simulink model "WaveStar"  (R2020b)
settings: Solver=ode4  StartTime=0  StopTime=141.2  FixedStep=0.001  MaxStep=0.001  RelTol=1e-3  EnableMultiTasking=on
values from neighbouring files (symbols this model uses):
  cc = 10.0    (= 10)    [controller_init.m]
  kc = 0    [controller_init.m]
  L_AB = 0.412    [controller_init.m]
  L_AC = 0.2    [controller_init.m]
  mc = 0    [controller_init.m]
  McSat = inf    [controller_init.m]
  simu = simulationClass()    [wecSimInputFile.m]
  xPcTs = 0.001    [controller_init.m]
undefined symbols (not defined in the file or in its folder): body, constraint, geometry, HPfreq, hydroData, LPfreq, pto, X, Y, Z
libraries: nesl_utility x36, sm_lib x26, WECSim_Lib_Body_Elements x5, simulink x2, WECSim_Lib_Constraints x2, WECSim_Lib_Frames x1
(part 2 of 2)

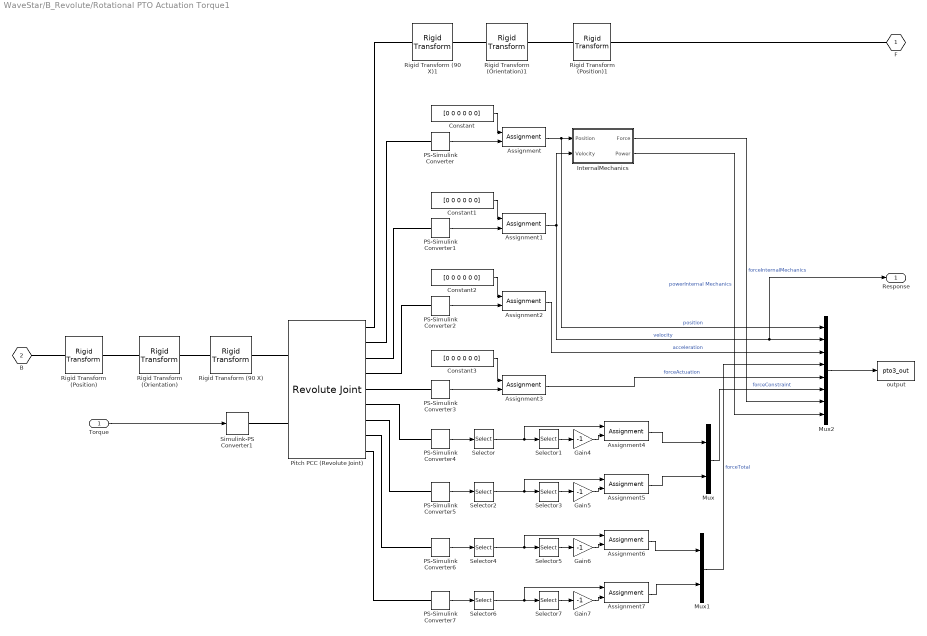
== system WaveStar/B_Revolute/Rotational PTO Actuation Torque1 ==
  Torque : Inport
  "Assignment " : Assignment  IndexOptions=Index vector (dialog)  Indices=5  OutputSizes=1
  Assignment1 : Assignment  IndexOptions=Index vector (dialog)  Indices=5  OutputSizes=1
  Assignment2 : Assignment  IndexOptions=Index vector (dialog)  Indices=5  OutputSizes=1
  Assignment3 : Assignment  IndexOptions=Index vector (dialog)  Indices=5  OutputSizes=1
  Assignment{4..7} (4 alike) : Assignment  DiagnosticForDimensions=Warning  IndexOptions=Index vector (dialog)  Indices=3  OutputSizes=1
  Constant{,1..3} (4 alike) : Constant  Value=[0 0 0 0 0 0]
  Gain{4..7} (4 alike) : Gain  Gain=-1
  InternalMechanics : Subsystem
  Mux : Mux  Inputs=2
  Mux1 : Mux  Inputs=2
  Mux2 : Mux  Inputs=8
  PS-Simulink Converter{,1..7} (8 alike) : nesl_utility/PS-Simulink Converter  PhysicalDomain=network_engine_domain  SubClassName=ps_output  LeftPortType=input  RightPortType=output  PseudoPeriodic=off  Frequencies=[]  VectorFormat=1-D array  Unit=1  AffineConversion=off
  Pitch PCC (Revolute Joint) : sm_lib/Joints/Revolute Joint  JointMode=Normal  SenseConstraintForce=on  SenseConstraintForceX=off  SenseConstraintForceY=off  SenseConstraintForceZ=off  SenseConstraintTorque=on  SenseConstraintTorqueX=off  SenseConstraintTorqueY=off  SenseConstraintTorqueZ=off  SenseTotalForce=on  SenseTotalForceX=off  SenseTotalForceY=off  SenseTotalForceZ=off  SenseTotalTorque=on  SenseTotalTorqueX=off  SenseTotalTorqueY=off  SenseTotalTorqueZ=off  CompositeWrenchDir=BaseOnFollower  CompositeWrenchFrame=BaseFrame  EquilibriumPosition=0  EquilibriumPositionUnits=deg  SpringStiffness=pto.stiffness  SpringStiffnessUnits=N*m/rad  DampingCoefficient=pto.damping  DampingCoefficientUnits=N*m/(rad/s)  TorqueActuationMode=InputTorque  MotionActuationMode=ComputedMotion  SensePosition=on  SenseVelocity=on  SenseAcceleration=on  SenseTorqueForce=on  SenseLowerLimitTorqueForce=off  SenseUpperLimitTorqueForce=off  LowerLimitSpecify=off  LowerLimitBound=-90  LowerLimitBoundUnits=deg  LowerLimitStiffness=1e4  LowerLimitStiffnessUnits=N*m/deg  LowerLimitDamping=10  LowerLimitDampingUnits=N*m/(deg/s)  LowerLimitTransitionRegionWidth=0.1  LowerLimitTransitionRegionWidthUnits=deg  UpperLimitSpecify=off  UpperLimitBound=90  UpperLimitBoundUnits=deg  UpperLimitStiffness=1e4  UpperLimitStiffnessUnits=N*m/deg  UpperLimitDamping=10  UpperLimitDampingUnits=N*m/(deg/s)  UpperLimitTransitionRegionWidth=0.1  UpperLimitTransitionRegionWidthUnits=deg  PositionTargetSpecify=off  PositionTargetPriority=High  PositionTargetValue=0  PositionTargetValueUnits=deg  VelocityTargetSpecify=off  VelocityTargetPriority=High  VelocityTargetValue=0  VelocityTargetValueUnits=deg/s
  Rigid Transform (Position) : sm_lib/Frames and Transforms/Rigid Transform  TranslationMethod=Cartesian  TranslationStandardOffset=0  TranslationStandardOffsetUnits=m  TranslationStandardAxis=+Z  TranslationCartesianOffset=pto.initial.displacement + pto.location  TranslationCartesianOffsetUnits=m  TranslationROffset=0  TranslationROffsetUnits=m  TranslationZOffset=0  TranslationZOffsetUnits=m  TranslationThetaOffset=0  TranslationThetaOffsetUnits=deg  RotationMethod=None  RotationAngleUnits=rad  RotationStandardAxis=+Y  RotationAngle=0  RotationArbitraryAxis=[0 1 0]  FollAlignAxisA=+X  BaseAlignAxisA=+Y  FollAlignAxisB=+Y  BaseAlignAxisB=+Z  RotationSequenceAxes=FollowerAxes  RotationSequence=XYX  RotationSequenceAngles=[0 0 0]  RotationSequenceAnglesUnits=deg  RotationMatrix=[1 0 0; 0 1 0; 0 0 1]  Quaternion=[1 0 0 0]
  Rigid Transform (Position)1 : sm_lib/Frames and Transforms/Rigid Transform  TranslationMethod=Cartesian  TranslationStandardOffset=0  TranslationStandardOffsetUnits=m  TranslationStandardAxis=+Z  TranslationCartesianOffset=pto.initial.displacement + pto.location  TranslationCartesianOffsetUnits=m  TranslationROffset=0  TranslationROffsetUnits=m  TranslationZOffset=0  TranslationZOffsetUnits=m  TranslationThetaOffset=0  TranslationThetaOffsetUnits=deg  RotationMethod=None  RotationAngleUnits=rad  RotationStandardAxis=+Y  RotationAngle=0  RotationArbitraryAxis=[0 1 0]  FollAlignAxisA=+X  BaseAlignAxisA=+Y  FollAlignAxisB=+Y  BaseAlignAxisB=+Z  RotationSequenceAxes=FollowerAxes  RotationSequence=XYX  RotationSequenceAngles=[0 0 0]  RotationSequenceAnglesUnits=deg  RotationMatrix=[1 0 0; 0 1 0; 0 0 1]  Quaternion=[1 0 0 0]
  Rigid Transform (90 X) : sm_lib/Frames and Transforms/Rigid Transform  TranslationMethod=None  TranslationStandardOffset=0  TranslationStandardOffsetUnits=m  TranslationStandardAxis=+Z  TranslationCartesianOffset=0  TranslationCartesianOffsetUnits=m  TranslationROffset=0  TranslationROffsetUnits=m  TranslationZOffset=0  TranslationZOffsetUnits=m  TranslationThetaOffset=0  TranslationThetaOffsetUnits=deg  RotationMethod=StandardAxis  RotationAngleUnits=deg  RotationStandardAxis=+X  RotationAngle=-90  RotationArbitraryAxis=[0 1 0]  FollAlignAxisA=+X  BaseAlignAxisA=+Y  FollAlignAxisB=+Y  BaseAlignAxisB=+Z  RotationSequenceAxes=FollowerAxes  RotationSequence=XYX  RotationSequenceAngles=[0 0 0]  RotationSequenceAnglesUnits=deg  RotationMatrix=[1 0 0; 0 1 0; 0 0 1]  Quaternion=[1 0 0 0]
  Rigid Transform (90 X)1 : sm_lib/Frames and Transforms/Rigid Transform  TranslationMethod=None  TranslationStandardOffset=0  TranslationStandardOffsetUnits=m  TranslationStandardAxis=+Z  TranslationCartesianOffset=0  TranslationCartesianOffsetUnits=m  TranslationROffset=0  TranslationROffsetUnits=m  TranslationZOffset=0  TranslationZOffsetUnits=m  TranslationThetaOffset=0  TranslationThetaOffsetUnits=deg  RotationMethod=StandardAxis  RotationAngleUnits=deg  RotationStandardAxis=+X  RotationAngle=-90  RotationArbitraryAxis=[0 1 0]  FollAlignAxisA=+X  BaseAlignAxisA=+Y  FollAlignAxisB=+Y  BaseAlignAxisB=+Z  RotationSequenceAxes=FollowerAxes  RotationSequence=XYX  RotationSequenceAngles=[0 0 0]  RotationSequenceAnglesUnits=deg  RotationMatrix=[1 0 0; 0 1 0; 0 0 1]  Quaternion=[1 0 0 0]
  Rigid Transform (Orientation) : sm_lib/Frames and Transforms/Rigid Transform  TranslationMethod=None  TranslationStandardOffset=0  TranslationStandardOffsetUnits=m  TranslationStandardAxis=+Z  TranslationCartesianOffset=0  TranslationCartesianOffsetUnits=m  TranslationROffset=0  TranslationROffsetUnits=m  TranslationZOffset=0  TranslationZOffsetUnits=m  TranslationThetaOffset=0  TranslationThetaOffsetUnits=deg  RotationMethod=RotationMatrix  RotationAngleUnits=rad  RotationStandardAxis=+Y  RotationAngle=0  RotationArbitraryAxis=[0 1 0]  FollAlignAxisA=+X  BaseAlignAxisA=+Y  FollAlignAxisB=+Y  BaseAlignAxisB=+Z  RotationSequenceAxes=FollowerAxes  RotationSequence=XYX  RotationSequenceAngles=[0 0 0]  RotationSequenceAnglesUnits=deg  RotationMatrix=pto.orientation.rotationMatrix  Quaternion=[1 0 0 0]
  Rigid Transform (Orientation)1 : sm_lib/Frames and Transforms/Rigid Transform  TranslationMethod=None  TranslationStandardOffset=0  TranslationStandardOffsetUnits=m  TranslationStandardAxis=+Z  TranslationCartesianOffset=0  TranslationCartesianOffsetUnits=m  TranslationROffset=0  TranslationROffsetUnits=m  TranslationZOffset=0  TranslationZOffsetUnits=m  TranslationThetaOffset=0  TranslationThetaOffsetUnits=deg  RotationMethod=RotationMatrix  RotationAngleUnits=rad  RotationStandardAxis=+Y  RotationAngle=0  RotationArbitraryAxis=[0 1 0]  FollAlignAxisA=+X  BaseAlignAxisA=+Y  FollAlignAxisB=+Y  BaseAlignAxisB=+Z  RotationSequenceAxes=FollowerAxes  RotationSequence=XYX  RotationSequenceAngles=[0 0 0]  RotationSequenceAnglesUnits=deg  RotationMatrix=pto.orientation.rotationMatrix  Quaternion=[1 0 0 0]
  Selector{,2,4,6} (4 alike) : Selector  InputPortWidth=3  IndexOptions=Index vector (dialog)  Indices=[1 3 2]  OutputSizes=1
  Selector{1,3,5,7} (4 alike) : Selector  InputPortWidth=3  IndexOptions=Index vector (dialog)  Indices=[3]  OutputSizes=1
  Simulink-PS Converter1 : nesl_utility/Simulink-PS Converter  PhysicalDomain=network_engine_domain  SubClassName=ps_input  LeftPortType=input  RightPortType=output  PseudoPeriodic=off  Frequencies=[]  NoiseDistribution=none  NoiseParameters=[]  Unit=1  AffineConversion=off  FilteringAndDerivatives=zero  SimscapeFilterOrder=1  InputFilterTimeConstant=0.001  UdotUserProvided=1
  output : ToWorkspace  VariableName=pto3_out  SaveFormat=Structure With Time  SampleTime=-1
      settings: Decimation=round(simu.dtOut/simu.dt,0)
  F : PMIOPort  Side=Right
  B : PMIOPort  Port=2  Side=Left
  Response : Outport  VectorParamsAs1DForOutWhenUnconnected=off
  wires:
  Torque/1 -> Simulink-PS Converter1/1
  "Assignment "/1 -> Mux2/1, InternalMechanics/1(Position)  "position"
  Assignment1/1 -> Response/1, Mux2/2, InternalMechanics/2(Velocity)  "velocity"
  Assignment2/1 -> Mux2/3  "acceleration"
  Selector2/1 -> Assignment5/1, Selector3/1
  Selector3/1 -> Gain5/1
  Gain5/1 -> Assignment5/2
  Selector/1 -> Assignment4/1, Selector1/1
  Selector1/1 -> Gain4/1
  Gain4/1 -> Assignment4/2
  Assignment5/1 -> Mux/2
  Assignment4/1 -> Mux/1
  Mux/1 -> Mux2/6  "forceConstraint"
  PS-Simulink Converter5/1 -> Selector2/1
  PS-Simulink Converter4/1 -> Selector/1
  Mux2/1 -> output/1
  Mux1/1 -> Mux2/4  "forceTotal"
  Selector6/1 -> Selector7/1, Assignment7/1
  Selector7/1 -> Gain7/1
  Gain7/1 -> Assignment7/2
  Selector4/1 -> Selector5/1, Assignment6/1
  Selector5/1 -> Gain6/1
  Gain6/1 -> Assignment6/2
  PS-Simulink Converter6/1 -> Selector4/1
  PS-Simulink Converter7/1 -> Selector6/1
  Assignment7/1 -> Mux1/2
  Assignment6/1 -> Mux1/1
  Constant/1 -> "Assignment "/1
  PS-Simulink Converter/1 -> "Assignment "/2
  Constant1/1 -> Assignment1/1
  PS-Simulink Converter1/1 -> Assignment1/2
  Constant2/1 -> Assignment2/1
  PS-Simulink Converter2/1 -> Assignment2/2
  Constant3/1 -> Assignment3/1
  PS-Simulink Converter3/1 -> Assignment3/2
  Assignment3/1 -> Mux2/5  "forceActuation"
  InternalMechanics/1(Force) -> Mux2/7  "forceInternalMechanics"
  InternalMechanics/2(Power) -> Mux2/8  "powerInternal Mechanics"
  connections:
  Rigid Transform (Position)1/LConn1 -- F/RConn1
  Rigid Transform (Position)/RConn1 -- Rigid Transform (Orientation)/LConn1
  Rigid Transform (Orientation)/RConn1 -- Rigid Transform (90 X)/LConn1
  Rigid Transform (Orientation)1/RConn1 -- Rigid Transform (90 X)1/LConn1
  Rigid Transform (Position)1/RConn1 -- Rigid Transform (Orientation)1/LConn1
  Rigid Transform (90 X)/RConn1 -- Pitch PCC (Revolute Joint)/LConn1
  Pitch PCC (Revolute Joint)/LConn2 -- Simulink-PS Converter1/RConn1
  Rigid Transform (Position)/LConn1 -- B/RConn1
  PS-Simulink Converter7/LConn1 -- Pitch PCC (Revolute Joint)/RConn9
  PS-Simulink Converter6/LConn1 -- Pitch PCC (Revolute Joint)/RConn8
  PS-Simulink Converter5/LConn1 -- Pitch PCC (Revolute Joint)/RConn7
  PS-Simulink Converter4/LConn1 -- Pitch PCC (Revolute Joint)/RConn6
  Pitch PCC (Revolute Joint)/RConn2 -- PS-Simulink Converter/LConn1
  Pitch PCC (Revolute Joint)/RConn3 -- PS-Simulink Converter1/LConn1
  PS-Simulink Converter2/LConn1 -- Pitch PCC (Revolute Joint)/RConn4
  PS-Simulink Converter3/LConn1 -- Pitch PCC (Revolute Joint)/RConn5
  Rigid Transform (90 X)1/RConn1 -- Pitch PCC (Revolute Joint)/RConn1

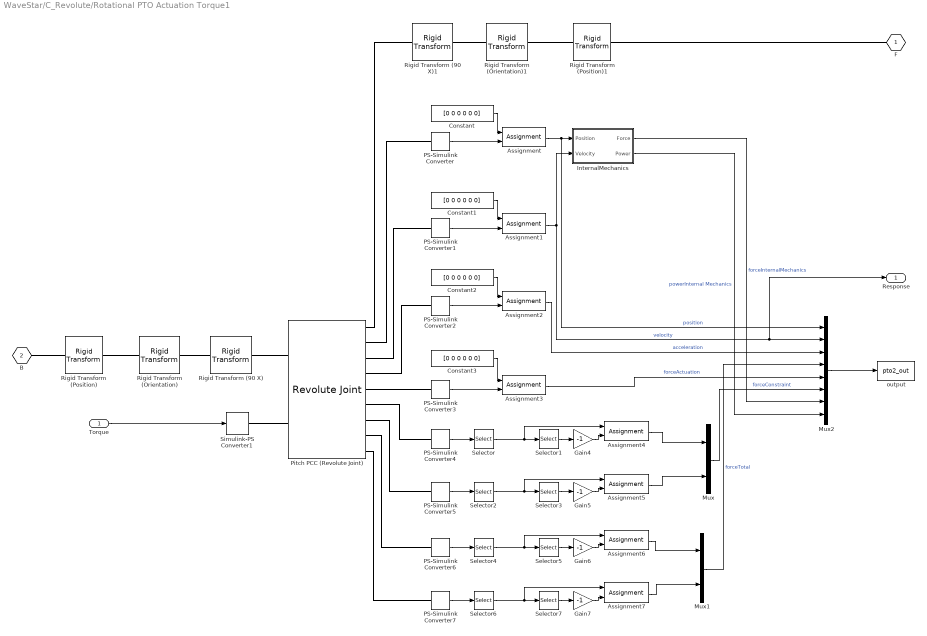
== system WaveStar/C_Revolute/Rotational PTO Actuation Torque1 ==
  Torque : Inport
  "Assignment " : Assignment  IndexOptions=Index vector (dialog)  Indices=5  OutputSizes=1
  Assignment1 : Assignment  IndexOptions=Index vector (dialog)  Indices=5  OutputSizes=1
  Assignment2 : Assignment  IndexOptions=Index vector (dialog)  Indices=5  OutputSizes=1
  Assignment3 : Assignment  IndexOptions=Index vector (dialog)  Indices=5  OutputSizes=1
  Assignment{4..7} (4 alike) : Assignment  DiagnosticForDimensions=Warning  IndexOptions=Index vector (dialog)  Indices=3  OutputSizes=1
  Constant{,1..3} (4 alike) : Constant  Value=[0 0 0 0 0 0]
  Gain{4..7} (4 alike) : Gain  Gain=-1
  InternalMechanics : Subsystem
  Mux : Mux  Inputs=2
  Mux1 : Mux  Inputs=2
  Mux2 : Mux  Inputs=8
  PS-Simulink Converter{,1..7} (8 alike) : nesl_utility/PS-Simulink Converter  PhysicalDomain=network_engine_domain  SubClassName=ps_output  LeftPortType=input  RightPortType=output  PseudoPeriodic=off  Frequencies=[]  VectorFormat=1-D array  Unit=1  AffineConversion=off
  Pitch PCC (Revolute Joint) : sm_lib/Joints/Revolute Joint  JointMode=Normal  SenseConstraintForce=on  SenseConstraintForceX=off  SenseConstraintForceY=off  SenseConstraintForceZ=off  SenseConstraintTorque=on  SenseConstraintTorqueX=off  SenseConstraintTorqueY=off  SenseConstraintTorqueZ=off  SenseTotalForce=on  SenseTotalForceX=off  SenseTotalForceY=off  SenseTotalForceZ=off  SenseTotalTorque=on  SenseTotalTorqueX=off  SenseTotalTorqueY=off  SenseTotalTorqueZ=off  CompositeWrenchDir=BaseOnFollower  CompositeWrenchFrame=BaseFrame  EquilibriumPosition=0  EquilibriumPositionUnits=deg  SpringStiffness=pto.stiffness  SpringStiffnessUnits=N*m/rad  DampingCoefficient=pto.damping  DampingCoefficientUnits=N*m/(rad/s)  TorqueActuationMode=InputTorque  MotionActuationMode=ComputedMotion  SensePosition=on  SenseVelocity=on  SenseAcceleration=on  SenseTorqueForce=on  SenseLowerLimitTorqueForce=off  SenseUpperLimitTorqueForce=off  LowerLimitSpecify=off  LowerLimitBound=-90  LowerLimitBoundUnits=deg  LowerLimitStiffness=1e4  LowerLimitStiffnessUnits=N*m/deg  LowerLimitDamping=10  LowerLimitDampingUnits=N*m/(deg/s)  LowerLimitTransitionRegionWidth=0.1  LowerLimitTransitionRegionWidthUnits=deg  UpperLimitSpecify=off  UpperLimitBound=90  UpperLimitBoundUnits=deg  UpperLimitStiffness=1e4  UpperLimitStiffnessUnits=N*m/deg  UpperLimitDamping=10  UpperLimitDampingUnits=N*m/(deg/s)  UpperLimitTransitionRegionWidth=0.1  UpperLimitTransitionRegionWidthUnits=deg  PositionTargetSpecify=off  PositionTargetPriority=High  PositionTargetValue=0  PositionTargetValueUnits=deg  VelocityTargetSpecify=off  VelocityTargetPriority=High  VelocityTargetValue=0  VelocityTargetValueUnits=deg/s
  Rigid Transform (Position) : sm_lib/Frames and Transforms/Rigid Transform  TranslationMethod=Cartesian  TranslationStandardOffset=0  TranslationStandardOffsetUnits=m  TranslationStandardAxis=+Z  TranslationCartesianOffset=pto.initial.displacement + pto.location  TranslationCartesianOffsetUnits=m  TranslationROffset=0  TranslationROffsetUnits=m  TranslationZOffset=0  TranslationZOffsetUnits=m  TranslationThetaOffset=0  TranslationThetaOffsetUnits=deg  RotationMethod=None  RotationAngleUnits=rad  RotationStandardAxis=+Y  RotationAngle=0  RotationArbitraryAxis=[0 1 0]  FollAlignAxisA=+X  BaseAlignAxisA=+Y  FollAlignAxisB=+Y  BaseAlignAxisB=+Z  RotationSequenceAxes=FollowerAxes  RotationSequence=XYX  RotationSequenceAngles=[0 0 0]  RotationSequenceAnglesUnits=deg  RotationMatrix=[1 0 0; 0 1 0; 0 0 1]  Quaternion=[1 0 0 0]
  Rigid Transform (Position)1 : sm_lib/Frames and Transforms/Rigid Transform  TranslationMethod=Cartesian  TranslationStandardOffset=0  TranslationStandardOffsetUnits=m  TranslationStandardAxis=+Z  TranslationCartesianOffset=pto.initial.displacement + pto.location  TranslationCartesianOffsetUnits=m  TranslationROffset=0  TranslationROffsetUnits=m  TranslationZOffset=0  TranslationZOffsetUnits=m  TranslationThetaOffset=0  TranslationThetaOffsetUnits=deg  RotationMethod=None  RotationAngleUnits=rad  RotationStandardAxis=+Y  RotationAngle=0  RotationArbitraryAxis=[0 1 0]  FollAlignAxisA=+X  BaseAlignAxisA=+Y  FollAlignAxisB=+Y  BaseAlignAxisB=+Z  RotationSequenceAxes=FollowerAxes  RotationSequence=XYX  RotationSequenceAngles=[0 0 0]  RotationSequenceAnglesUnits=deg  RotationMatrix=[1 0 0; 0 1 0; 0 0 1]  Quaternion=[1 0 0 0]
  Rigid Transform (90 X) : sm_lib/Frames and Transforms/Rigid Transform  TranslationMethod=None  TranslationStandardOffset=0  TranslationStandardOffsetUnits=m  TranslationStandardAxis=+Z  TranslationCartesianOffset=0  TranslationCartesianOffsetUnits=m  TranslationROffset=0  TranslationROffsetUnits=m  TranslationZOffset=0  TranslationZOffsetUnits=m  TranslationThetaOffset=0  TranslationThetaOffsetUnits=deg  RotationMethod=StandardAxis  RotationAngleUnits=deg  RotationStandardAxis=+X  RotationAngle=-90  RotationArbitraryAxis=[0 1 0]  FollAlignAxisA=+X  BaseAlignAxisA=+Y  FollAlignAxisB=+Y  BaseAlignAxisB=+Z  RotationSequenceAxes=FollowerAxes  RotationSequence=XYX  RotationSequenceAngles=[0 0 0]  RotationSequenceAnglesUnits=deg  RotationMatrix=[1 0 0; 0 1 0; 0 0 1]  Quaternion=[1 0 0 0]
  Rigid Transform (90 X)1 : sm_lib/Frames and Transforms/Rigid Transform  TranslationMethod=None  TranslationStandardOffset=0  TranslationStandardOffsetUnits=m  TranslationStandardAxis=+Z  TranslationCartesianOffset=0  TranslationCartesianOffsetUnits=m  TranslationROffset=0  TranslationROffsetUnits=m  TranslationZOffset=0  TranslationZOffsetUnits=m  TranslationThetaOffset=0  TranslationThetaOffsetUnits=deg  RotationMethod=StandardAxis  RotationAngleUnits=deg  RotationStandardAxis=+X  RotationAngle=-90  RotationArbitraryAxis=[0 1 0]  FollAlignAxisA=+X  BaseAlignAxisA=+Y  FollAlignAxisB=+Y  BaseAlignAxisB=+Z  RotationSequenceAxes=FollowerAxes  RotationSequence=XYX  RotationSequenceAngles=[0 0 0]  RotationSequenceAnglesUnits=deg  RotationMatrix=[1 0 0; 0 1 0; 0 0 1]  Quaternion=[1 0 0 0]
  Rigid Transform (Orientation) : sm_lib/Frames and Transforms/Rigid Transform  TranslationMethod=None  TranslationStandardOffset=0  TranslationStandardOffsetUnits=m  TranslationStandardAxis=+Z  TranslationCartesianOffset=0  TranslationCartesianOffsetUnits=m  TranslationROffset=0  TranslationROffsetUnits=m  TranslationZOffset=0  TranslationZOffsetUnits=m  TranslationThetaOffset=0  TranslationThetaOffsetUnits=deg  RotationMethod=RotationMatrix  RotationAngleUnits=rad  RotationStandardAxis=+Y  RotationAngle=0  RotationArbitraryAxis=[0 1 0]  FollAlignAxisA=+X  BaseAlignAxisA=+Y  FollAlignAxisB=+Y  BaseAlignAxisB=+Z  RotationSequenceAxes=FollowerAxes  RotationSequence=XYX  RotationSequenceAngles=[0 0 0]  RotationSequenceAnglesUnits=deg  RotationMatrix=pto.orientation.rotationMatrix  Quaternion=[1 0 0 0]
  Rigid Transform (Orientation)1 : sm_lib/Frames and Transforms/Rigid Transform  TranslationMethod=None  TranslationStandardOffset=0  TranslationStandardOffsetUnits=m  TranslationStandardAxis=+Z  TranslationCartesianOffset=0  TranslationCartesianOffsetUnits=m  TranslationROffset=0  TranslationROffsetUnits=m  TranslationZOffset=0  TranslationZOffsetUnits=m  TranslationThetaOffset=0  TranslationThetaOffsetUnits=deg  RotationMethod=RotationMatrix  RotationAngleUnits=rad  RotationStandardAxis=+Y  RotationAngle=0  RotationArbitraryAxis=[0 1 0]  FollAlignAxisA=+X  BaseAlignAxisA=+Y  FollAlignAxisB=+Y  BaseAlignAxisB=+Z  RotationSequenceAxes=FollowerAxes  RotationSequence=XYX  RotationSequenceAngles=[0 0 0]  RotationSequenceAnglesUnits=deg  RotationMatrix=pto.orientation.rotationMatrix  Quaternion=[1 0 0 0]
  Selector{,2,4,6} (4 alike) : Selector  InputPortWidth=3  IndexOptions=Index vector (dialog)  Indices=[1 3 2]  OutputSizes=1
  Selector{1,3,5,7} (4 alike) : Selector  InputPortWidth=3  IndexOptions=Index vector (dialog)  Indices=[3]  OutputSizes=1
  Simulink-PS Converter1 : nesl_utility/Simulink-PS Converter  PhysicalDomain=network_engine_domain  SubClassName=ps_input  LeftPortType=input  RightPortType=output  PseudoPeriodic=off  Frequencies=[]  NoiseDistribution=none  NoiseParameters=[]  Unit=1  AffineConversion=off  FilteringAndDerivatives=zero  SimscapeFilterOrder=1  InputFilterTimeConstant=0.001  UdotUserProvided=1
  output : ToWorkspace  VariableName=pto2_out  SaveFormat=Structure With Time  SampleTime=-1
      settings: Decimation=round(simu.dtOut/simu.dt,0)
  F : PMIOPort  Side=Right
  B : PMIOPort  Port=2  Side=Left
  Response : Outport  VectorParamsAs1DForOutWhenUnconnected=off
  wires:
  Torque/1 -> Simulink-PS Converter1/1
  "Assignment "/1 -> Mux2/1, InternalMechanics/1(Position)  "position"
  Assignment1/1 -> Response/1, Mux2/2, InternalMechanics/2(Velocity)  "velocity"
  Assignment2/1 -> Mux2/3  "acceleration"
  Selector2/1 -> Assignment5/1, Selector3/1
  Selector3/1 -> Gain5/1
  Gain5/1 -> Assignment5/2
  Selector/1 -> Assignment4/1, Selector1/1
  Selector1/1 -> Gain4/1
  Gain4/1 -> Assignment4/2
  Assignment5/1 -> Mux/2
  Assignment4/1 -> Mux/1
  Mux/1 -> Mux2/6  "forceConstraint"
  PS-Simulink Converter5/1 -> Selector2/1
  PS-Simulink Converter4/1 -> Selector/1
  Mux2/1 -> output/1
  Mux1/1 -> Mux2/4  "forceTotal"
  Selector6/1 -> Selector7/1, Assignment7/1
  Selector7/1 -> Gain7/1
  Gain7/1 -> Assignment7/2
  Selector4/1 -> Selector5/1, Assignment6/1
  Selector5/1 -> Gain6/1
  Gain6/1 -> Assignment6/2
  PS-Simulink Converter6/1 -> Selector4/1
  PS-Simulink Converter7/1 -> Selector6/1
  Assignment7/1 -> Mux1/2
  Assignment6/1 -> Mux1/1
  Constant/1 -> "Assignment "/1
  PS-Simulink Converter/1 -> "Assignment "/2
  Constant1/1 -> Assignment1/1
  PS-Simulink Converter1/1 -> Assignment1/2
  Constant2/1 -> Assignment2/1
  PS-Simulink Converter2/1 -> Assignment2/2
  Constant3/1 -> Assignment3/1
  PS-Simulink Converter3/1 -> Assignment3/2
  Assignment3/1 -> Mux2/5  "forceActuation"
  InternalMechanics/1(Force) -> Mux2/7  "forceInternalMechanics"
  InternalMechanics/2(Power) -> Mux2/8  "powerInternal Mechanics"
  connections:
  Rigid Transform (Position)1/LConn1 -- F/RConn1
  Rigid Transform (Position)/RConn1 -- Rigid Transform (Orientation)/LConn1
  Rigid Transform (Orientation)/RConn1 -- Rigid Transform (90 X)/LConn1
  Rigid Transform (Orientation)1/RConn1 -- Rigid Transform (90 X)1/LConn1
  Rigid Transform (Position)1/RConn1 -- Rigid Transform (Orientation)1/LConn1
  Rigid Transform (90 X)/RConn1 -- Pitch PCC (Revolute Joint)/LConn1
  Pitch PCC (Revolute Joint)/LConn2 -- Simulink-PS Converter1/RConn1
  Rigid Transform (Position)/LConn1 -- B/RConn1
  PS-Simulink Converter7/LConn1 -- Pitch PCC (Revolute Joint)/RConn9
  PS-Simulink Converter6/LConn1 -- Pitch PCC (Revolute Joint)/RConn8
  PS-Simulink Converter5/LConn1 -- Pitch PCC (Revolute Joint)/RConn7
  PS-Simulink Converter4/LConn1 -- Pitch PCC (Revolute Joint)/RConn6
  Pitch PCC (Revolute Joint)/RConn2 -- PS-Simulink Converter/LConn1
  Pitch PCC (Revolute Joint)/RConn3 -- PS-Simulink Converter1/LConn1
  PS-Simulink Converter2/LConn1 -- Pitch PCC (Revolute Joint)/RConn4
  PS-Simulink Converter3/LConn1 -- Pitch PCC (Revolute Joint)/RConn5
  Rigid Transform (90 X)1/RConn1 -- Pitch PCC (Revolute Joint)/RConn1

== system WaveStar/Controller/Linear ==
  wave_gauge_1 : Inport
  wave_gauge_2 : Inport  Port=2
  wave_gauge_3 : Inport  Port=3
  float_accel : Inport  Port=4
  motor_force : Inport  Port=5
  "motor_pos " : Inport  Port=6
  WECCCOMP Controller : Subsystem
  cmd_force : Outport  VectorParamsAs1DForOutWhenUnconnected=off
  wires:
  WECCCOMP Controller/1(cmd_force) -> cmd_force/1
  float_accel/1 -> WECCCOMP Controller/1(float_accel_rot)
  motor_force/1 -> WECCCOMP Controller/2(motor_force)
  "motor_pos "/1 -> WECCCOMP Controller/3("motor_pos ")
  wave_gauge_1/1 -> WECCCOMP Controller/4(wave_gauge_1)
  wave_gauge_2/1 -> WECCCOMP Controller/5(wave_gauge_2)
  wave_gauge_3/1 -> WECCCOMP Controller/6(wave_gauge_3)

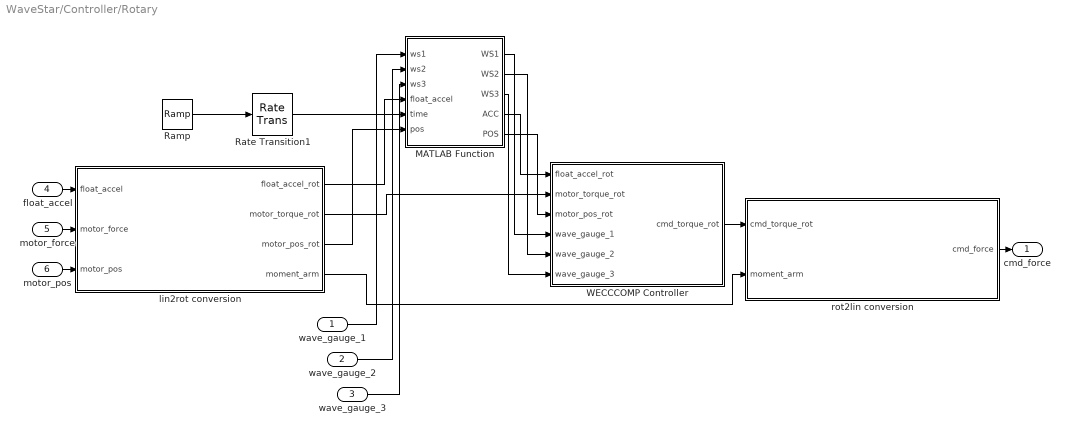
== system WaveStar/Controller/Rotary ==
  wave_gauge_1 : Inport
  wave_gauge_2 : Inport  Port=2
  wave_gauge_3 : Inport  Port=3
  float_accel : Inport  Port=4
  motor_force : Inport  Port=5
  "motor_pos " : Inport  Port=6
  MATLAB Function : MATLAB Function  TreatAsAtomicUnit=on
  Ramp : simulink/Sources/Ramp  slope=1  start=0  InitialOutput=0
  Rate Transition1 : RateTransition  OutPortSampleTime=simu.dt
  WECCCOMP Controller : Subsystem
  lin2rot conversion : Subsystem
  rot2lin conversion : Subsystem
  cmd_force : Outport  VectorParamsAs1DForOutWhenUnconnected=off
  wires:
  float_accel/1 -> lin2rot conversion/1(float_accel)
  motor_force/1 -> lin2rot conversion/2(motor_force)
  "motor_pos "/1 -> lin2rot conversion/3("motor_pos ")
  rot2lin conversion/1(cmd_force) -> cmd_force/1
  WECCCOMP Controller/1(cmd_torque_rot) -> rot2lin conversion/1(cmd_torque_rot)
  lin2rot conversion/2(motor_torque_rot) -> WECCCOMP Controller/2(motor_torque_rot)
  lin2rot conversion/1("float_accel_rot ") -> MATLAB Function/4(float_accel)
  lin2rot conversion/3(motor_pos_rot) -> MATLAB Function/6(pos)
  wave_gauge_1/1 -> MATLAB Function/1(ws1)
  lin2rot conversion/4(moment_arm) -> rot2lin conversion/2(moment_arm)
  wave_gauge_2/1 -> MATLAB Function/2(ws2)
  wave_gauge_3/1 -> MATLAB Function/3(ws3)
  MATLAB Function/1(WS1) -> WECCCOMP Controller/4(wave_gauge_1)
  MATLAB Function/2(WS2) -> WECCCOMP Controller/5(wave_gauge_2)
  MATLAB Function/3(WS3) -> WECCCOMP Controller/6(wave_gauge_3)
  MATLAB Function/4(ACC) -> WECCCOMP Controller/1(float_accel_rot)
  MATLAB Function/5(POS) -> WECCCOMP Controller/3("motor_pos_rot ")
  Ramp/1 -> Rate Transition1/1
  Rate Transition1/1 -> MATLAB Function/5(time)

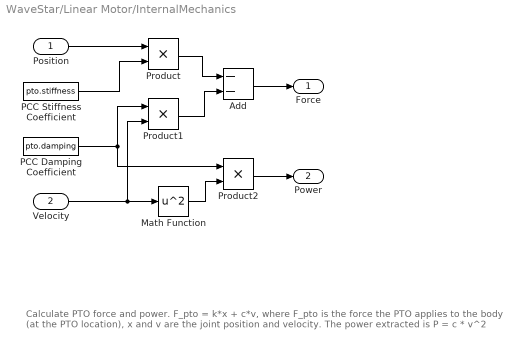
== system WaveStar/Linear Motor/InternalMechanics ==
  note: Calculate PTO force and power.
      |
      | F_pto  = k*x + c*v,
      | where F_pto is the force the PTO applies to the body (at the PTO location), x and v are the joint position and velocity.
      |
      | The power extracted is
      | P = c * v^2
  Position : Inport
  Velocity : Inport  Port=2
  Add : Sum  Inputs=--
  Math Function : Math  Operator=square  SignedPower=on  SaturateOnIntegerOverflow=on
  PCC Damping Coefficient : Constant  Value=pto.damping
  PCC Stiffness Coefficient : Constant  Value=pto.stiffness
  Product : Product  Inputs=**
  Product1 : Product  Inputs=**
  Product2 : Product  Inputs=**
  Force : Outport  VectorParamsAs1DForOutWhenUnconnected=off
  Power : Outport  Port=2  VectorParamsAs1DForOutWhenUnconnected=off
  wires:
  PCC Damping Coefficient/1 -> Product1/1, Product2/1
  Product2/1 -> Power/1
  Velocity/1 -> Math Function/1, Product1/2
  PCC Stiffness Coefficient/1 -> Product/2
  Position/1 -> Product/1
  Add/1 -> Force/1
  Math Function/1 -> Product2/2
  Product/1 -> Add/1
  Product1/1 -> Add/2

== system WaveStar/A_Revolute/Rotational PTO Actuation Torque1/InternalMechanics ==
  note: Calculate PTO force and power.
      |
      | F_pto  = k*x + c*v,
      | where F_pto is the force the PTO applies to the body (at the PTO location), x and v are the joint position and velocity.
      |
      | The power extracted is
      | P_pto = F_pto * v
  Position : Inport
  Velocity : Inport  Port=2
  Add : Sum  Inputs=--
  PCC Damping Coefficient : Constant  Value=pto.damping
  PCC Stiffness Coefficient : Constant  Value=pto.stiffness
  Product : Product  Inputs=**
  Product1 : Product  Inputs=**
  Product2 : Product  Inputs=**
  Force : Outport  VectorParamsAs1DForOutWhenUnconnected=off
  Power : Outport  Port=2  VectorParamsAs1DForOutWhenUnconnected=off
  wires:
  PCC Damping Coefficient/1 -> Product1/1
  Product2/1 -> Power/1
  PCC Stiffness Coefficient/1 -> Product/2
  Position/1 -> Product/1
  Add/1 -> Force/1, Product2/1
  Velocity/1 -> Product1/2, Product2/2
  Product/1 -> Add/1
  Product1/1 -> Add/2

== system WaveStar/B_Revolute/Rotational PTO Actuation Torque1/InternalMechanics ==
  note: Calculate PTO force and power.
      |
      | F_pto  = k*x + c*v,
      | where F_pto is the force the PTO applies to the body (at the PTO location), x and v are the joint position and velocity.
      |
      | The power extracted is
      | P_pto = F_pto * v
  Position : Inport
  Velocity : Inport  Port=2
  Add : Sum  Inputs=--
  PCC Damping Coefficient : Constant  Value=pto.damping
  PCC Stiffness Coefficient : Constant  Value=pto.stiffness
  Product : Product  Inputs=**
  Product1 : Product  Inputs=**
  Product2 : Product  Inputs=**
  Force : Outport  VectorParamsAs1DForOutWhenUnconnected=off
  Power : Outport  Port=2  VectorParamsAs1DForOutWhenUnconnected=off
  wires:
  PCC Damping Coefficient/1 -> Product1/1
  Product2/1 -> Power/1
  PCC Stiffness Coefficient/1 -> Product/2
  Position/1 -> Product/1
  Add/1 -> Force/1, Product2/1
  Velocity/1 -> Product1/2, Product2/2
  Product/1 -> Add/1
  Product1/1 -> Add/2

== system WaveStar/C_Revolute/Rotational PTO Actuation Torque1/InternalMechanics ==
  note: Calculate PTO force and power.
      |
      | F_pto  = k*x + c*v,
      | where F_pto is the force the PTO applies to the body (at the PTO location), x and v are the joint position and velocity.
      |
      | The power extracted is
      | P_pto = F_pto * v
  Position : Inport
  Velocity : Inport  Port=2
  Add : Sum  Inputs=--
  PCC Damping Coefficient : Constant  Value=pto.damping
  PCC Stiffness Coefficient : Constant  Value=pto.stiffness
  Product : Product  Inputs=**
  Product1 : Product  Inputs=**
  Product2 : Product  Inputs=**
  Force : Outport  VectorParamsAs1DForOutWhenUnconnected=off
  Power : Outport  Port=2  VectorParamsAs1DForOutWhenUnconnected=off
  wires:
  PCC Damping Coefficient/1 -> Product1/1
  Product2/1 -> Power/1
  PCC Stiffness Coefficient/1 -> Product/2
  Position/1 -> Product/1
  Add/1 -> Force/1, Product2/1
  Velocity/1 -> Product1/2, Product2/2
  Product/1 -> Add/1
  Product1/1 -> Add/2

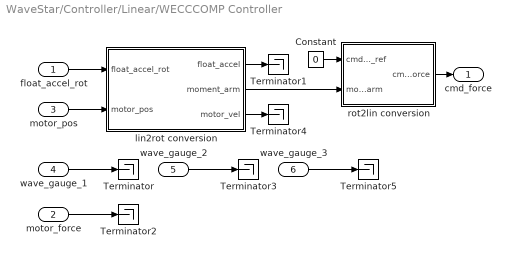
== system WaveStar/Controller/Linear/WECCCOMP Controller ==
  float_accel_rot : Inport
  motor_force : Inport  Port=2
  "motor_pos " : Inport  Port=3
  wave_gauge_1 : Inport  Port=4
  wave_gauge_2 : Inport  Port=5
  wave_gauge_3 : Inport  Port=6
  Constant : Constant  Value=0
  Terminator{,1..5} (6 alike) : Terminator
  lin2rot conversion : Subsystem
  rot2lin conversion : Subsystem
  cmd_force : Outport  VectorParamsAs1DForOutWhenUnconnected=off
  wires:
  lin2rot conversion/2(moment_arm) -> rot2lin conversion/2(moment_arm)
  wave_gauge_1/1 -> Terminator/1
  "motor_pos "/1 -> lin2rot conversion/2("motor_pos ")
  motor_force/1 -> Terminator2/1
  float_accel_rot/1 -> lin2rot conversion/1(float_accel_rot)
  rot2lin conversion/1(cmd_force) -> cmd_force/1
  Constant/1 -> rot2lin conversion/1(cmd_force_ref)
  lin2rot conversion/1("float_accel ") -> Terminator1/1
  lin2rot conversion/3(motor_vel) -> Terminator4/1
  wave_gauge_2/1 -> Terminator3/1
  wave_gauge_3/1 -> Terminator5/1

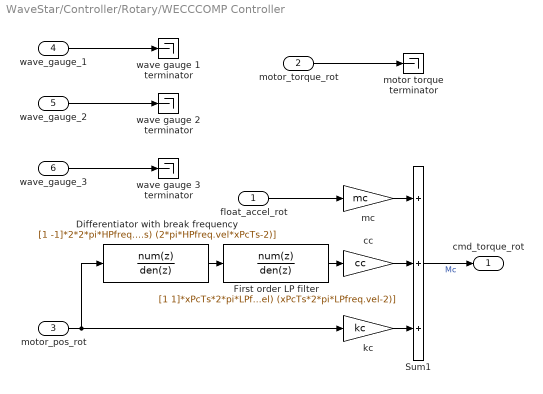
== system WaveStar/Controller/Rotary/WECCCOMP Controller ==
  float_accel_rot : Inport
  motor_torque_rot : Inport  Port=2
  "motor_pos_rot " : Inport  Port=3
  wave_gauge_1 : Inport  Port=4
  wave_gauge_2 : Inport  Port=5
  wave_gauge_3 : Inport  Port=6
  Differentiator with break frequency : DiscreteTransferFcn  Numerator=[1 -1]*2*2*pi*HPfreq.vel  Denominator=[(2+2*pi*HPfreq.vel*xPcTs) (2*pi*HPfreq.vel*xPcTs-2)]
  First order LP filter : DiscreteTransferFcn  Numerator=[1 1]*xPcTs*2*pi*LPfreq.vel  Denominator=[(2+xPcTs*2*pi*LPfreq.vel) (xPcTs*2*pi*LPfreq.vel-2)]
  Sum1 : Sum  Inputs=+++
  cc : Gain  Gain=cc
  kc : Gain  Gain=kc
  mc : Gain  Gain=mc
  motor torque terminator : Terminator
  wave gauge 1 terminator : Terminator
  wave gauge 2 terminator : Terminator
  wave gauge 3 terminator : Terminator
  cmd_torque_rot : Outport  VectorParamsAs1DForOutWhenUnconnected=off
  wires:
  cc/1 -> Sum1/2
  kc/1 -> Sum1/3
  "motor_pos_rot "/1 -> Differentiator with break frequency/1, kc/1
  float_accel_rot/1 -> mc/1
  mc/1 -> Sum1/1
  motor_torque_rot/1 -> motor torque terminator/1
  wave_gauge_1/1 -> wave gauge 1 terminator/1
  Differentiator with break frequency/1 -> First order LP filter/1
  First order LP filter/1 -> cc/1
  Sum1/1 -> cmd_torque_rot/1  "Mc"
  wave_gauge_2/1 -> wave gauge 2 terminator/1
  wave_gauge_3/1 -> wave gauge 3 terminator/1

== system WaveStar/Controller/Rotary/lin2rot conversion ==
  float_accel : Inport
  motor_force : Inport  Port=2
  "motor_pos " : Inport  Port=3
  Axial Motor Force : Selector  InputPortWidth=6  IndexOptions=Index vector (dialog)  Indices=[3]  OutputSizes=1
  Axial Position : Selector  InputPortWidth=6  IndexOptions=Index vector (dialog)  Indices=[3]  OutputSizes=1
  Divide => K (m)2 : Product  Inputs=**
  Linear2Angular Conversion : Subsystem
  "float_accel_rot " : Outport  VectorParamsAs1DForOutWhenUnconnected=off
  motor_torque_rot : Outport  Port=2  VectorParamsAs1DForOutWhenUnconnected=off
  motor_pos_rot : Outport  Port=3  VectorParamsAs1DForOutWhenUnconnected=off
  moment_arm : Outport  Port=4  VectorParamsAs1DForOutWhenUnconnected=off
  wires:
  "motor_pos "/1 -> Axial Position/1
  Linear2Angular Conversion/2(moment_arm) -> Divide => K (m)2/1, moment_arm/1
  Axial Position/1 -> Linear2Angular Conversion/1(x_cyl)
  Linear2Angular Conversion/1(Theta) -> motor_pos_rot/1
  float_accel/1 -> "float_accel_rot "/1  "Angular Acceleration"
  motor_force/1 -> Axial Motor Force/1
  Axial Motor Force/1 -> Divide => K (m)2/2
  Divide => K (m)2/1 -> motor_torque_rot/1

== system WaveStar/Controller/Rotary/rot2lin conversion ==
  cmd_torque_rot : Inport
  moment_arm : Inport  Port=2
  Cmd torque to measured torque dynamics : DiscreteTransferFcn  Numerator="[0.96294775   -1.92342278    0.96053421]"  Denominator="[1.00000000   -1.99777700    0.99783206]"
  "Divide " : Product  Inputs=*/
  Gain : Gain  Gain=-1
  Saturation : Saturate  UpperLimit=McSat  LowerLimit=-McSat
  cmd_force : Outport  VectorParamsAs1DForOutWhenUnconnected=off
  wires:
  "Divide "/1 -> cmd_force/1
  moment_arm/1 -> "Divide "/2
  Saturation/1 -> Gain/1  "Mc_sat"
  Gain/1 -> "Divide "/1
  cmd_torque_rot/1 -> Cmd torque to measured torque dynamics/1
  Cmd torque to measured torque dynamics/1 -> Saturation/1

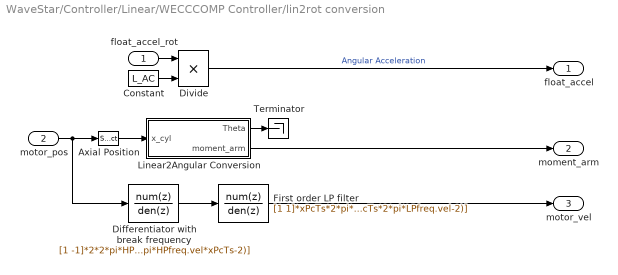
== system WaveStar/Controller/Linear/WECCCOMP Controller/lin2rot conversion ==
  float_accel_rot : Inport
  "motor_pos " : Inport  Port=2
  Axial Position : Selector  InputPortWidth=6  IndexOptions=Index vector (dialog)  Indices=[3]  OutputSizes=1
  Constant : Constant  Value=L_AC
  Differentiator with break frequency : DiscreteTransferFcn  Numerator=[1 -1]*2*2*pi*HPfreq.vel  Denominator=[(2+2*pi*HPfreq.vel*xPcTs) (2*pi*HPfreq.vel*xPcTs-2)]
  Divide : Product  Inputs=**
  First order LP filter : DiscreteTransferFcn  Numerator=[1 1]*xPcTs*2*pi*LPfreq.vel  Denominator=[(2+xPcTs*2*pi*LPfreq.vel) (xPcTs*2*pi*LPfreq.vel-2)]
  Linear2Angular Conversion : Subsystem
  Terminator : Terminator
  "float_accel " : Outport  VectorParamsAs1DForOutWhenUnconnected=off
  moment_arm : Outport  Port=2  VectorParamsAs1DForOutWhenUnconnected=off
  motor_vel : Outport  Port=3  VectorParamsAs1DForOutWhenUnconnected=off
  wires:
  "motor_pos "/1 -> Differentiator with break frequency/1, Axial Position/1
  Linear2Angular Conversion/2(moment_arm) -> moment_arm/1
  Axial Position/1 -> Linear2Angular Conversion/1(x_cyl)
  Linear2Angular Conversion/1(Theta) -> Terminator/1
  float_accel_rot/1 -> Divide/1
  Constant/1 -> Divide/2
  Divide/1 -> "float_accel "/1  "Angular Acceleration"
  Differentiator with break frequency/1 -> First order LP filter/1
  First order LP filter/1 -> motor_vel/1

== system WaveStar/Controller/Linear/WECCCOMP Controller/rot2lin conversion ==
  cmd_force_ref : Inport
  moment_arm : Inport  Port=2
  "Divide " : Product  Inputs=*/
  Gain : Gain  Gain=-1
  Multiply : Product  Inputs=**
  Saturation : Saturate  UpperLimit=McSat  LowerLimit=-McSat
  comand torque to measured torque dynamics : DiscreteTransferFcn  Numerator="[ 0.9821   -1.9618    0.9797]"  Denominator="[1.0000   -1.9978    0.9978]"
  cmd_force : Outport  VectorParamsAs1DForOutWhenUnconnected=off
  wires:
  "Divide "/1 -> cmd_force/1
  moment_arm/1 -> Multiply/2, "Divide "/2
  Saturation/1 -> Gain/1  "Mc_sat"
  Gain/1 -> "Divide "/1
  comand torque to measured torque dynamics/1 -> Saturation/1
  cmd_force_ref/1 -> Multiply/1
  Multiply/1 -> comand torque to measured torque dynamics/1

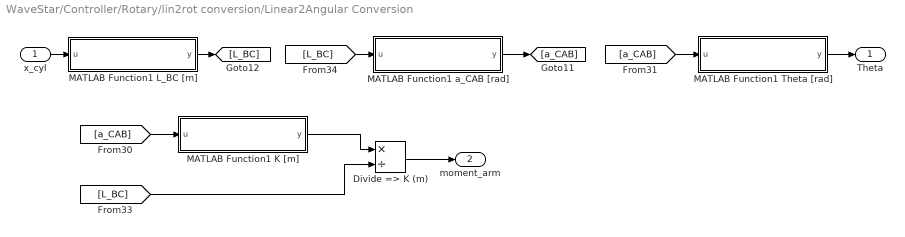
== system WaveStar/Controller/Rotary/lin2rot conversion/Linear2Angular Conversion ==
  x_cyl : Inport
  Divide => K (m) : Product  Inputs=*/
  MATLAB Function1 K [m] : MATLAB Function  TreatAsAtomicUnit=on
  MATLAB Function1 L_BC [m] : MATLAB Function  TreatAsAtomicUnit=on
  MATLAB Function1 Theta [rad] : MATLAB Function  TreatAsAtomicUnit=on
  MATLAB Function1 a_CAB [rad] : MATLAB Function  TreatAsAtomicUnit=on
  Theta : Outport  VectorParamsAs1DForOutWhenUnconnected=off
  moment_arm : Outport  Port=2  VectorParamsAs1DForOutWhenUnconnected=off
  wires:
  MATLAB Function1 L_BC [m]/1(y) -> [L_BC]
  [a_CAB] -> MATLAB Function1 Theta [rad]/1(u)
  MATLAB Function1 K [m]/1(y) -> Divide => K (m)/1
  [L_BC] -> MATLAB Function1 a_CAB [rad]/1(u)
  [L_BC] -> Divide => K (m)/2
  x_cyl/1 -> MATLAB Function1 L_BC [m]/1(u)
  Divide => K (m)/1 -> moment_arm/1
  MATLAB Function1 a_CAB [rad]/1(y) -> [a_CAB]
  [a_CAB] -> MATLAB Function1 K [m]/1(u)
  MATLAB Function1 Theta [rad]/1(y) -> Theta/1

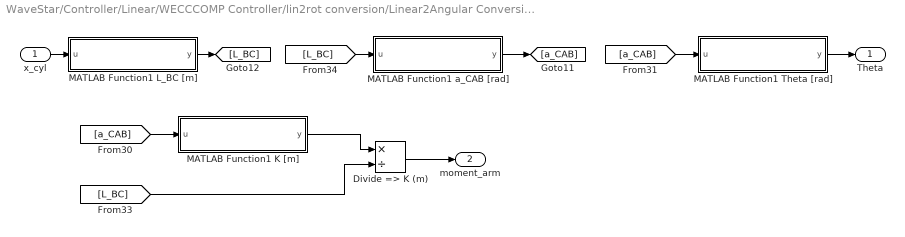
== system WaveStar/Controller/Linear/WECCCOMP Controller/lin2rot conversion/Linear2Angular Conversion ==
  x_cyl : Inport
  Divide => K (m) : Product  Inputs=*/
  MATLAB Function1 K [m] : MATLAB Function  TreatAsAtomicUnit=on
  MATLAB Function1 L_BC [m] : MATLAB Function  TreatAsAtomicUnit=on
  MATLAB Function1 Theta [rad] : MATLAB Function  TreatAsAtomicUnit=on
  MATLAB Function1 a_CAB [rad] : MATLAB Function  TreatAsAtomicUnit=on
  Theta : Outport  VectorParamsAs1DForOutWhenUnconnected=off
  moment_arm : Outport  Port=2  VectorParamsAs1DForOutWhenUnconnected=off
  wires:
  MATLAB Function1 L_BC [m]/1(y) -> [L_BC]
  [a_CAB] -> MATLAB Function1 Theta [rad]/1(u)
  MATLAB Function1 K [m]/1(y) -> Divide => K (m)/1
  [L_BC] -> MATLAB Function1 a_CAB [rad]/1(u)
  [L_BC] -> Divide => K (m)/2
  x_cyl/1 -> MATLAB Function1 L_BC [m]/1(u)
  Divide => K (m)/1 -> moment_arm/1
  MATLAB Function1 a_CAB [rad]/1(y) -> [a_CAB]
  [a_CAB] -> MATLAB Function1 K [m]/1(u)
  MATLAB Function1 Theta [rad]/1(y) -> Theta/1

== matlab function WaveStar/A_Revolute/MATLAB Function ==
  data: time input; vel input; t output; brkwy_trq parameter double; brkwy_vel parameter double; Col_trq parameter double; visc_coef parameter double
function t = friction(time,vel,brkwy_trq, brkwy_vel, Col_trq, visc_coef)
    w = -vel(5);

    %{
    brkwy_trq = .25;         % Breakaway friction torque
    brkwy_vel = 0.1;        % Breakaway friction velocity
    Col_trq = .20;           % Coulomb friction torque
    visc_coef = 0.001;      % Viscous friction coefficient
    %}
    
    static_scale = sqrt(2*exp(1))*(brkwy_trq-Col_trq);  % Scale factor for static torque
    static_thr = sqrt(2)*brkwy_vel;                     % Velocity threshold for static torque
    Col_thr = brkwy_vel/10;                             % Velocity threshold for Coulomb torque
    
    if (55 < time)&&(time < 115)
    t = visc_coef * w ...
         + static_scale * (w/static_thr*exp(-(w/static_thr)^2)) ...
         + Col_trq * tanh(w/Col_thr);
    else
        t = 0;
    end
end

%{
parameters
    brkwy_trq = { 25, 'N*m' };          % Breakaway friction torque
    brkwy_vel = { 0.1, 'rad/s' };       % Breakaway friction velocity
    Col_trq = { 20, 'N*m' };            % Coulomb friction torque
    visc_coef = { 0.001, 'N*m*s/rad' }; % Viscous friction coefficient
end

parameters (Access=private)
    static_scale = sqrt(2*exp(1))*(brkwy_trq-Col_trq);  % Scale factor for static torque
    static_thr = sqrt(2)*brkwy_vel;                     % Velocity threshold for static torque
    Col_thr = brkwy_vel/10;                             % Velocity threshold for Coulomb torque
end

equations
    % Parameter range checking
    assert(brkwy_trq>0)
    assert(brkwy_vel>0)
    assert(Col_trq>0)
    assert(Col_trq<=brkwy_trq)
    assert(visc_coef>=0)
    % Torque is a combination of viscous, static, and Coulomb losses
    t == visc_coef * w ...
         + static_scale * (w/static_thr*exp(-(w/static_thr)^2)) ...
         + Col_trq * tanh(w/Col_thr);
end
%}

== matlab function WaveStar/Controller/Rotary/lin2rot conversion/Linear2Angular Conversion/MATLAB Function1 L_BC [m] ==
  data: u input; y output; L_BC_neutral parameter
 function y = fcn(u,L_BC_neutral)
%#codegen
%
y = u+L_BC_neutral';

== matlab function WaveStar/Controller/Rotary/lin2rot conversion/Linear2Angular Conversion/MATLAB Function1 Theta [rad] ==
  data: u input; y output; a_CAB_neutral parameter
function y = fcn(u,a_CAB_neutral)
%#codegen
y = u-a_CAB_neutral';

== matlab function WaveStar/Controller/Rotary/lin2rot conversion/Linear2Angular Conversion/MATLAB Function1 a_CAB [rad] ==
  data: u input; y output; L_AB parameter; L_AC parameter
function y = fcn(u,L_AB,L_AC)
%#codegen
%
y = acos((u.^2-L_AB'^2-L_AC'^2)/(-2*L_AB'*L_AC'));

== matlab function WaveStar/Controller/Linear/WECCCOMP Controller/lin2rot conversion/Linear2Angular Conversion/MATLAB Function1 K [m] ==
  data: u input; y output; L_AB parameter; L_AC parameter
function y = fcn(u,L_AB,L_AC)
%#codegen
y = L_AB'*L_AC'*sin(u);

== matlab function WaveStar/Controller/Linear/WECCCOMP Controller/lin2rot conversion/Linear2Angular Conversion/MATLAB Function1 L_BC [m] ==
  data: u input; y output; L_BC_neutral parameter
 function y = fcn(u,L_BC_neutral)
%#codegen
%
y = u+L_BC_neutral';

== matlab function WaveStar/Controller/Linear/WECCCOMP Controller/lin2rot conversion/Linear2Angular Conversion/MATLAB Function1 Theta [rad] ==
  data: u input; y output; a_CAB_neutral parameter
function y = fcn(u,a_CAB_neutral)
%#codegen
y = u-a_CAB_neutral';

== matlab function WaveStar/Controller/Rotary/lin2rot conversion/Linear2Angular Conversion/MATLAB Function1 K [m] ==
  data: u input; y output; L_AB parameter; L_AC parameter
function y = fcn(u,L_AB,L_AC)
%#codegen
y = L_AB'*L_AC'*sin(u);

== matlab function WaveStar/Controller/Linear/WECCCOMP Controller/lin2rot conversion/Linear2Angular Conversion/MATLAB Function1 a_CAB [rad] ==
  data: u input; y output; L_AB parameter; L_AC parameter
function y = fcn(u,L_AB,L_AC)
%#codegen
%
y = acos((u.^2-L_AB'^2-L_AC'^2)/(-2*L_AB'*L_AC'));

== matlab function WaveStar/C_Revolute/MATLAB Function ==
  data: vel input; t output; brkwy_trq parameter double; brkwy_vel parameter double; Col_trq parameter double; visc_coef parameter double
function t = friction(vel,brkwy_trq, brkwy_vel, Col_trq, visc_coef)
    w = -vel(5);

    %{
    brkwy_trq = .25;         % Breakaway friction torque
    brkwy_vel = 0.1;        % Breakaway friction velocity
    Col_trq = .20;           % Coulomb friction torque
    visc_coef = 0.001;      % Viscous friction coefficient
    %}
    
    static_scale = sqrt(2*exp(1))*(brkwy_trq-Col_trq);  % Scale factor for static torque
    static_thr = sqrt(2)*brkwy_vel;                     % Velocity threshold for static torque
    Col_thr = brkwy_vel/10;                             % Velocity threshold for Coulomb torque
    
    t = visc_coef * w ...
         + static_scale * (w/static_thr*exp(-(w/static_thr)^2)) ...
         + Col_trq * tanh(w/Col_thr);
end

%{
parameters
    brkwy_trq = { 25, 'N*m' };          % Breakaway friction torque
    brkwy_vel = { 0.1, 'rad/s' };       % Breakaway friction velocity
    Col_trq = { 20, 'N*m' };            % Coulomb friction torque
    visc_coef = { 0.001, 'N*m*s/rad' }; % Viscous friction coefficient
end

parameters (Access=private)
    static_scale = sqrt(2*exp(1))*(brkwy_trq-Col_trq);  % Scale factor for static torque
    static_thr = sqrt(2)*brkwy_vel;                     % Velocity threshold for static torque
    Col_thr = brkwy_vel/10;                             % Velocity threshold for Coulomb torque
end

equations
    % Parameter range checking
    assert(brkwy_trq>0)
    assert(brkwy_vel>0)
    assert(Col_trq>0)
    assert(Col_trq<=brkwy_trq)
    assert(visc_coef>=0)
    % Torque is a combination of viscous, static, and Coulomb losses
    t == visc_coef * w ...
         + static_scale * (w/static_thr*exp(-(w/static_thr)^2)) ...
         + Col_trq * tanh(w/Col_thr);
end
%}

== matlab function WaveStar/B_Revolute/MATLAB Function ==
  data: vel input; t output; brkwy_trq parameter double; brkwy_vel parameter double; Col_trq parameter double; visc_coef parameter double
function t = friction(vel,brkwy_trq, brkwy_vel, Col_trq, visc_coef)
    w = -vel(5);

    %{
    brkwy_trq = .25;         % Breakaway friction torque
    brkwy_vel = 0.1;        % Breakaway friction velocity
    Col_trq = .20;           % Coulomb friction torque
    visc_coef = 0.001;      % Viscous friction coefficient
    %}
    
    static_scale = sqrt(2*exp(1))*(brkwy_trq-Col_trq);  % Scale factor for static torque
    static_thr = sqrt(2)*brkwy_vel;                     % Velocity threshold for static torque
    Col_thr = brkwy_vel/10;                             % Velocity threshold for Coulomb torque
    
    t = visc_coef * w ...
         + static_scale * (w/static_thr*exp(-(w/static_thr)^2)) ...
         + Col_trq * tanh(w/Col_thr);
end

%{
parameters
    brkwy_trq = { 25, 'N*m' };          % Breakaway friction torque
    brkwy_vel = { 0.1, 'rad/s' };       % Breakaway friction velocity
    Col_trq = { 20, 'N*m' };            % Coulomb friction torque
    visc_coef = { 0.001, 'N*m*s/rad' }; % Viscous friction coefficient
end

parameters (Access=private)
    static_scale = sqrt(2*exp(1))*(brkwy_trq-Col_trq);  % Scale factor for static torque
    static_thr = sqrt(2)*brkwy_vel;                     % Velocity threshold for static torque
    Col_thr = brkwy_vel/10;                             % Velocity threshold for Coulomb torque
end

equations
    % Parameter range checking
    assert(brkwy_trq>0)
    assert(brkwy_vel>0)
    assert(Col_trq>0)
    assert(Col_trq<=brkwy_trq)
    assert(visc_coef>=0)
    % Torque is a combination of viscous, static, and Coulomb losses
    t == visc_coef * w ...
         + static_scale * (w/static_thr*exp(-(w/static_thr)^2)) ...
         + Col_trq * tanh(w/Col_thr);
end
%}

== matlab function WaveStar/Controller/Rotary/MATLAB Function ==
  data: ws1 input; WS1 output; ws2 input; ws3 input; float_accel input; WS2 output; WS3 output; ACC output; time input; pos input; POS output
function [WS1,WS2,WS3,ACC,POS] = addfault(ws1, ws2, ws3, float_accel, time, pos)
 
%% Wave Gauge 1
bias = 0;
drift = 0;
pDrop = 0.2; %0.3;
x = rand;
rn = 0.002*randn; %0.002*randn;
if x<pDrop
    WS1 = 0;
else
    WS1 = ws1+bias+drift*time+rn;
end
 
%% Wave Gauge 2
bias = 0;
drift = 0;
pDrop = 0.18; %0.15;
x = rand;
rn = 0.002*randn; %0.002*randn;
if x<pDrop
    WS2 = 0;
else
    WS2 = ws2+bias+drift*time+rn;
end

 
%% Wave Gauge 3
bias = 0;
drift = 0;
pDrop = 0.15; %0.2;
x = rand;
rn = 0.002*randn; %0.002*randn;
if x<pDrop
    WS3 = 0;
else
    WS3 = ws3+bias+drift*time+rn;
end
 
%% Accelerometer
bias = 0;
drift = 0;
pDrop = 0.08; %0.23;
x = rand;
rn = 0.25*randn; %0.25*randn;
if x<pDrop
    ACC = 0;
else
    ACC = float_accel+bias+drift*time+rn;
end

%% Position
bias = 0;
drift = 0;
pDrop = 0.03; %0.01;
x = rand;
rn = 0.003*randn; %0.003*randn;

if x<pDrop
    POS = 0;
else
    POS = pos+bias+drift*time+rn;
end
